simulink model "prosjektoppgave"  (R2026a)
settings: Solver=VariableStepAuto  StopTime=100
values from neighbouring files (symbols this model uses):
  A = pi*(r)^2    (= 0.785398163397)    [linearsimple.m]
  At = pi*(rt)^2    (= 0.0176714586764)    [linearsimple.m]
  Atut = At/2    (= 0.00883572933822)    [linearsimple.m]
  g = 9.80665    [linearsimple.m]
  gammaverdi = -0.025    [linearsimple.m]
  h = 1    [linearsimple.m]
  h10 = 0.8*h    (= 0.8)    [linearsimple.m]
  h20 = 0.5*h    (= 0.5)    [linearsimple.m]
  hf = 0*h    (= 0)    [linearsimple.m]
  href = 0.7    [linearsimple.m]
  Kd = (2*zeta*omega_0+gamma-a)/d    [linearsimple.m]
  Ki = gamma*omega_0^2/d    [linearsimple.m]
  Kp = (omega_0^2+2*gamma*zeta*omega_0-b)/d    [linearsimple.m]
  L = 0.1    [linearsimple.m]
  n = 2    [linearsimple.m]
  omega_0 = 0.4    [linearsimple.m]
  p = 1000    [linearsimple.m]
  r = 0.5    [linearsimple.m]
  rt = 0.075    [linearsimple.m]
  sin_Amp = sqrt(2*g*h)*At/(n*A)    [linearsimple.m]
  Tau = (sqrt(0.11)+L)*sqrt(2*h/g)    [linearsimple.m]
  zeta = 1    [linearsimple.m]
libraries: sl_discontinuities x15, simulink x5, vrlib x1
settings Model: PacingRate=5  Creator=User  LastModifiedBy=User

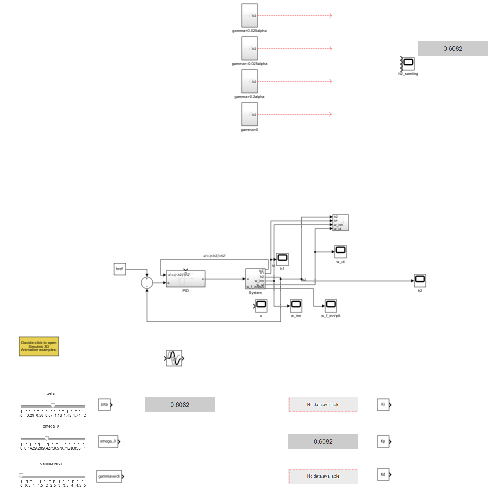
[thumbnail: Simulink's stored preview of the top-level diagram]
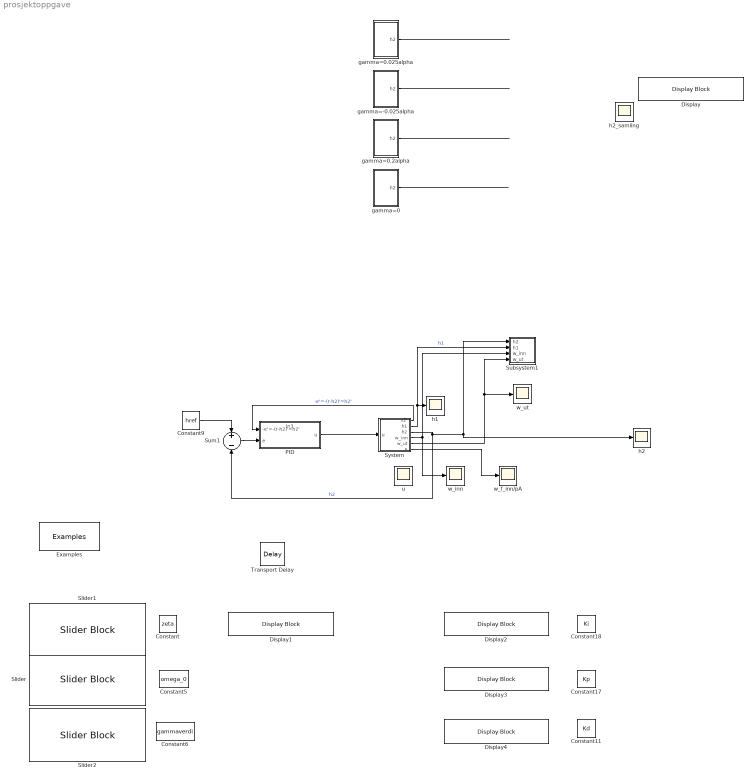
== system prosjektoppgave ==
  Constant : Constant  Value=zeta
  Constant11 : Constant  Value=Kd
  Constant17 : Constant  Value=Kp
  Constant18 : Constant  Value=Ki
  Constant5 : Constant  Value=omega_0
  Constant6 : Constant  Value=gammaverdi
  Constant9 : Constant  Value=href
  Display{,1..4} (5 alike) : DisplayBlock  LabelPosition=Hide  Transparency=1  GridColor=[0.502, 0.502, 0.502]
  Examples : vrlib/Examples
  PID : Subsystem
      settings: PortSchema="{\"entries\":[{\"content\":{\"sides\":[{\"content\":{\"connectorIds\":[\"In1\",\"In2\"]},\"type\":\"ConnectorPlacement.EquallySpacedRectSide\",\"uuid\":\"a96bb270-c3ec-4d15-9d6f-f29e3225f3c7\"},{\"content\":{\"connectorIds\":[\"Out1\"],\"side\":\"RIGHT\"},\"type\":\"ConnectorPlacement.EquallySpacedRectSide\",\"uuid\":\"f81bc953-5898-4b84-af0e-e30d44fc4639\"},{\"content\":{\"connectorIds\":[\"In3\"],\"side\":\"TOP\"},\"type\":\"ConnectorPlacement.EquallySpacedRectSide\",\"uuid\":\"08859213-698d-4bac-9d9f-733d026c3d6d\"}]},\"type\":\"ConnectorPlacement.EquallySpacedConnector\",\"uuid\":\"f15bc02d-61e9-4385-84d3-03e59a963aad\"}],\"packageUris\":[\"http://schema.mathworks.com/mf0/Connector/R2020b\"],\"version\":\"1.0\"}"
  Slider : SliderBlock  ScaleMax=1
  Slider1 : SliderBlock  ScaleMax=2
  Slider2 : SliderBlock  ScaleMax=5
  Subsystem1 : Subsystem
  Sum1 : Sum  Inputs=+-
  System : Subsystem
  Transport Delay : TransportDelay  DelayTime=Tau
  gamma=-0.025alpha : Subsystem
  gamma=0 : Subsystem
  gamma=0.025alpha : Subsystem
  gamma=0.2alpha : Subsystem
  h1 : Scope
      settings: ActiveDisplayYMinimum=0.74477697248915231  ActiveDisplayYMaximum=0.94477697248915227  DataLoggingVariableName=ScopeData6  DataLoggingSaveFormat=Array
  h2 : Scope
      settings: ActiveDisplayYMinimum=-0.00622784608789678  ActiveDisplayYMaximum=0.056050614791071034  DataLoggingVariableName=ScopeData11  DataLoggingSaveFormat=Array
  h2_samling : Scope  NumInputPorts=4
      settings: ActiveDisplayYMinimum=0.47019185858883861  ActiveDisplayYMaximum=0.76827327270045265  DataLoggingSaveFormat=Array
  u : Scope
      settings: ActiveDisplayYMinimum=-0.011988918852401206  ActiveDisplayYMaximum=0.078937646859600419  DataLoggingVariableName=ScopeData7  DataLoggingSaveFormat=Array
  w_f_inn/pA : Scope
      settings: ActiveDisplayYMinimum=-48.913386971378607  ActiveDisplayYMaximum=48.913374805426372  DataLoggingVariableName=ScopeData8  DataLoggingSaveFormat=Array
  w_inn : Scope
      settings: ActiveDisplayYMinimum=-9.7826777587122287  ActiveDisplayYMaximum=88.044099828410069  DataLoggingVariableName=ScopeData9  DataLoggingSaveFormat=Array
  w_ut : Scope
      settings: ActiveDisplayYMinimum=-0.00622784608789678  ActiveDisplayYMaximum=0.056050614791071034  DataLoggingVariableName=ScopeData10  DataLoggingSaveFormat=Array
  wires:
  gamma=0.025alpha/1(h2) -> ?
  gamma=-0.025alpha/1(h2) -> ?
  gamma=0.2alpha/1(h2) -> ?
  gamma=0/1(h2) -> ?
  System/4(w_inn) -> w_inn/1, Subsystem1/3(w_inn)
  Constant9/1 -> Sum1/1
  System/3(h2) -> h2/1, Subsystem1/1(h2), Sum1/2  "h2"
  System/2(h1) -> Subsystem1/2(h1), h1/1  "h1"
  System/5(w_ut) -> Subsystem1/4(w_ut), w_ut/1
  PID/1(u) -> System/1(u)
  System/6(w_f_inn/pA) -> w_f_inn/pA/1
  Sum1/1 -> PID/2(e)
  System/1(h2') -> PID/1(-e'=-(r-h2)'=h2')  "-e'=-(r-h2)'=h2'"

== system prosjektoppgave/PID ==
  -e'=-(r-h2)'=h2' : Inport
  e : Inport  Port=2
  In3 : Inport  Port=3
  Gain : Gain  Gain=1.2997
  Gain1 : Gain  Gain=-4.5681
  Gain2 : Gain  Gain=0.0126
  Integrator : Integrator
  Sum : Sum  Inputs=+++
  u : Outport
  wires:
  Integrator/1 -> Gain2/1
  Gain/1 -> Sum/2
  e/1 -> Gain/1, Integrator/1
  Gain2/1 -> Sum/3
  Gain1/1 -> Sum/1
  Sum/1 -> u/1
  -e'=-(r-h2)'=h2'/1 -> Gain1/1

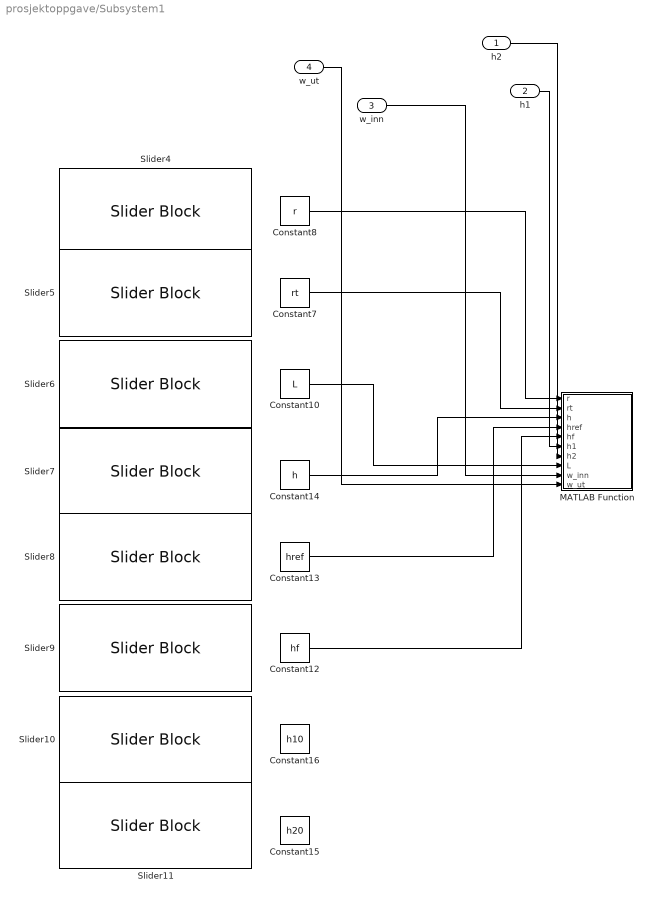
== system prosjektoppgave/Subsystem1 ==
  h2 : Inport
  h1 : Inport  Port=2
  w_inn : Inport  Port=3
  w_ut : Inport  Port=4
  Constant10 : Constant  Value=L
  Constant12 : Constant  Value=hf
  Constant13 : Constant  Value=href
  Constant14 : Constant  Value=h
  Constant15 : Constant  Value=h20
  Constant16 : Constant  Value=h10
  Constant7 : Constant  Value=rt
  Constant8 : Constant  Value=r
  MATLAB Function : MATLAB Function  TreatAsAtomicUnit=on
  Slider{4..5,10..11} (4 alike) : SliderBlock
  Slider{6..9} (4 alike) : SliderBlock  ScaleMax=1
  wires:
  h2/1 -> MATLAB Function/7(h2)
  Constant13/1 -> MATLAB Function/4(href)
  Constant10/1 -> MATLAB Function/8(L)
  Constant14/1 -> MATLAB Function/3(h)
  h1/1 -> MATLAB Function/6(h1)
  Constant12/1 -> MATLAB Function/5(hf)
  Constant8/1 -> MATLAB Function/1(r)
  Constant7/1 -> MATLAB Function/2(rt)
  w_inn/1 -> MATLAB Function/9(w_inn)
  w_ut/1 -> MATLAB Function/10(w_ut)

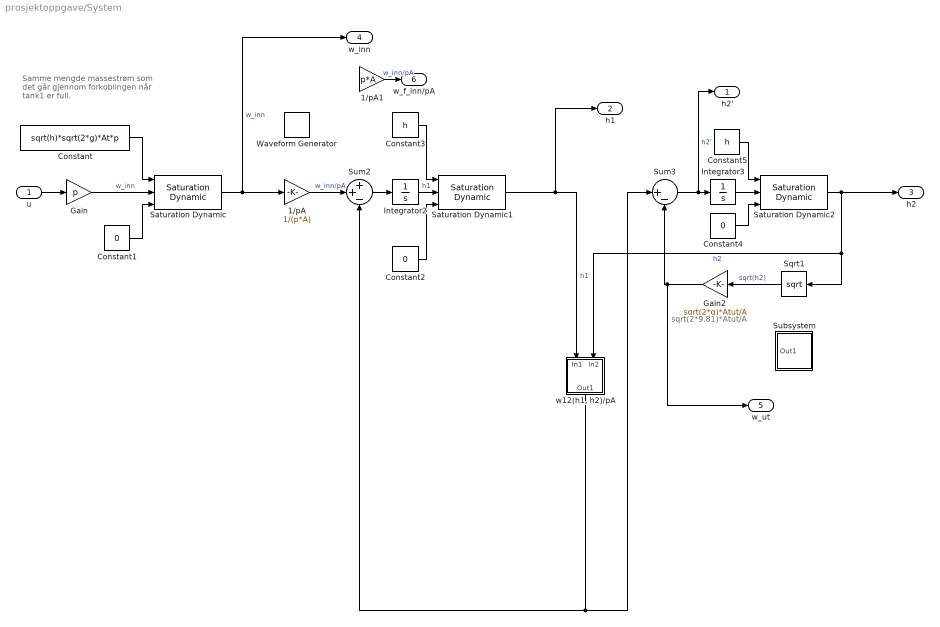
== system prosjektoppgave/System ==
  note: Samme mengde massestrøm
      | som det går gjennom
      | forkoblingen når tank1 er full.
  note: sqrt(2*9.81)*Atut/A
  u : Inport  OutMin=0
  1/pA : Gain  Gain=1/(p*A)
  1/pA1 : Gain  Gain=p*A
  Constant : Constant  Value=sqrt(h)*sqrt(2*g)*At*p
  Constant1 : Constant  Value=0
  Constant2 : Constant  Value=0
  Constant3 : Constant  Value=h
  Constant4 : Constant  Value=0
  Constant5 : Constant  Value=h
  Gain : Gain  Gain=p
  Gain2 : Gain  Gain=sqrt(2*g)*Atut/A
  Integrator2 : Integrator  InitialCondition=h10
  Integrator3 : Integrator  InitialCondition=h20
  Saturation Dynamic : sl_discontinuities/Saturation Dynamic  OutMin=[]  OutMax=[]  OutDataTypeStr=Inherit: Same as second input  OutDataType=fixdt(1, 16)  OutScaling=2^-10  DoSatur=off
      settings: LibrarySourceBlock=|
      | simulink/Discontinuities/Saturation
      | Dynamic
  Saturation Dynamic1 : sl_discontinuities/Saturation Dynamic  OutMin=[]  OutMax=[]  OutDataTypeStr=Inherit: Same as second input  OutDataType=fixdt(1, 16)  OutScaling=2^-10  DoSatur=off
      settings: LibrarySourceBlock=|
      | simulink/Discontinuities/Saturation
      | Dynamic
  Saturation Dynamic2 : sl_discontinuities/Saturation Dynamic  OutMin=[]  OutMax=[]  OutDataTypeStr=Inherit: Same as second input  OutDataType=fixdt(1, 16)  OutScaling=2^-10  DoSatur=off
      settings: LibrarySourceBlock=|
      | simulink/Discontinuities/Saturation
      | Dynamic
  Sqrt1 : Sqrt
  Subsystem : Subsystem
  Sum2 : Sum  Inputs=++-
  Sum3 : Sum  Inputs=|+-
  Waveform Generator : simulink/Sources/Waveform Generator  OutMin=0  OutMax=sqrt(2*g)*At/(n*A)  OutDataTypeStr=double  SelectedSignal=1  Signals=sin(sin_Amp, 0.025, 0)  BlockNames=MultiportSwitch_05447e85ab52467  SampleTime=0.1
  "w12(h1, h2)/pA" : Subsystem
  h2' : Outport  VectorParamsAs1DForOutWhenUnconnected=off
  h1 : Outport  Port=2
  h2 : Outport  Port=3
  w_inn : Outport  Port=4
  w_ut : Outport  Port=5
  w_f_inn/pA : Outport  Port=6
  wires:
  Sum2/1 -> Integrator2/1
  Sum3/1 -> h2'/1, Integrator3/1  "h2'"
  Constant1/1 -> Saturation Dynamic/3
  Constant/1 -> Saturation Dynamic/1
  Integrator2/1 -> Saturation Dynamic1/2  "h1"
  Saturation Dynamic1/1 -> "w12(h1, h2)/pA"/1(In1), h1/1  "h1"
  Constant2/1 -> Saturation Dynamic1/3
  Constant3/1 -> Saturation Dynamic1/1
  Integrator3/1 -> Saturation Dynamic2/2
  Saturation Dynamic2/1 -> Sqrt1/1, "w12(h1, h2)/pA"/2(In2), h2/1  "h2"
  Constant4/1 -> Saturation Dynamic2/3
  Constant5/1 -> Saturation Dynamic2/1
  u/1 -> Gain/1
  Gain/1 -> Saturation Dynamic/2  "w_inn"
  Saturation Dynamic/1 -> w_inn/1, 1/pA/1  "w_inn"
  1/pA/1 -> Sum2/2  "w_inn/pA"
  ? -> 1/pA1/1, Sum2/1  "w_f_inn/pA"
  "w12(h1, h2)/pA"/1(Out1) -> Sum3/1, Sum2/3
  Sqrt1/1 -> Gain2/1  "sqrt(h2)"
  1/pA1/1 -> w_f_inn/pA/1  "w_inn/pA"
  Gain2/1 -> w_ut/1, Sum3/2

== system prosjektoppgave/gamma=-0.025alpha ==
  Constant9 : Constant  Value=href
  PID : Subsystem
  Subsystem1 : Subsystem
  Sum1 : Sum  Inputs=+-
  System : Subsystem
  h1 : Scope
      settings: ActiveDisplayYMinimum=0.74477697248915231  ActiveDisplayYMaximum=0.94477697248915227  DataLoggingVariableName=ScopeData2  DataLoggingSaveFormat=Array
  u : Scope
      settings: ActiveDisplayYMinimum=-0.011988918852401206  ActiveDisplayYMaximum=0.078937646859600419  DataLoggingVariableName=ScopeData4  DataLoggingSaveFormat=Array
  w_f_inn/pA : Scope
      settings: ActiveDisplayYMinimum=-48.913386971378607  ActiveDisplayYMaximum=48.913374805426372  DataLoggingVariableName=ScopeData5  DataLoggingSaveFormat=Array
  w_inn : Scope
      settings: ActiveDisplayYMinimum=-9.7826777587122287  ActiveDisplayYMaximum=88.044099828410069  DataLoggingSaveFormat=Array
  w_ut : Scope
      settings: ActiveDisplayYMinimum=-0.00622784608789678  ActiveDisplayYMaximum=0.056050614791071034  DataLoggingVariableName=ScopeData3  DataLoggingSaveFormat=Array
  h2 : Outport
  wires:
  System/3(h2) -> h2/1, Subsystem1/1(h2), Sum1/2  "h2"
  System/4(w_inn) -> w_inn/1, Subsystem1/3(w_inn)
  System/5(w_ut) -> Subsystem1/4(w_ut), w_ut/1
  System/2(h1) -> Subsystem1/2(h1), h1/1  "h1"
  Sum1/1 -> PID/2(e)
  Constant9/1 -> Sum1/1
  System/1(h2') -> PID/1(-e'=-(r-h2)'=h2')  "-e'=-(r-h2)'=h2'"
  System/6(w_f_inn/pA) -> w_f_inn/pA/1
  PID/1(u) -> System/1(u)

== system prosjektoppgave/gamma=0 ==
  Constant9 : Constant  Value=href
  PID : Subsystem
  Subsystem1 : Subsystem
  Sum1 : Sum  Inputs=+-
  System : Subsystem
  h1 : Scope
      settings: ActiveDisplayYMinimum=0.74477697248915231  ActiveDisplayYMaximum=0.94477697248915227  DataLoggingVariableName=ScopeData2  DataLoggingSaveFormat=Array
  u : Scope
      settings: ActiveDisplayYMinimum=-0.011988918852401206  ActiveDisplayYMaximum=0.078937646859600419  DataLoggingVariableName=ScopeData4  DataLoggingSaveFormat=Array
  w_f_inn/pA : Scope
      settings: ActiveDisplayYMinimum=-48.913386971378607  ActiveDisplayYMaximum=48.913374805426372  DataLoggingVariableName=ScopeData5  DataLoggingSaveFormat=Array
  w_inn : Scope
      settings: ActiveDisplayYMinimum=-9.7826777587122287  ActiveDisplayYMaximum=88.044099828410069  DataLoggingSaveFormat=Array
  w_ut : Scope
      settings: ActiveDisplayYMinimum=-0.00622784608789678  ActiveDisplayYMaximum=0.056050614791071034  DataLoggingVariableName=ScopeData3  DataLoggingSaveFormat=Array
  h2 : Outport
  wires:
  System/3(h2) -> h2/1, Subsystem1/1(h2), Sum1/2  "h2"
  System/4(w_inn) -> w_inn/1, Subsystem1/3(w_inn)
  System/5(w_ut) -> Subsystem1/4(w_ut), w_ut/1
  System/2(h1) -> Subsystem1/2(h1), h1/1  "h1"
  Sum1/1 -> PID/2(e)
  Constant9/1 -> Sum1/1
  System/1(h2') -> PID/1(-e'=-(r-h2)'=h2')  "-e'=-(r-h2)'=h2'"
  System/6(w_f_inn/pA) -> w_f_inn/pA/1
  PID/1(u) -> System/1(u)

== system prosjektoppgave/gamma=0.025alpha ==
  Constant9 : Constant  Value=href
  PID : Subsystem
  Subsystem1 : Subsystem
  Sum1 : Sum  Inputs=+-
  System : Subsystem
  h1 : Scope
      settings: ActiveDisplayYMinimum=0.74477697248915231  ActiveDisplayYMaximum=0.94477697248915227  DataLoggingVariableName=ScopeData2  DataLoggingSaveFormat=Array
  u : Scope
      settings: ActiveDisplayYMinimum=-0.011988918852401206  ActiveDisplayYMaximum=0.078937646859600419  DataLoggingVariableName=ScopeData4  DataLoggingSaveFormat=Array
  w_f_inn/pA : Scope
      settings: ActiveDisplayYMinimum=-48.913386971378607  ActiveDisplayYMaximum=48.913374805426372  DataLoggingVariableName=ScopeData5  DataLoggingSaveFormat=Array
  w_inn : Scope
      settings: ActiveDisplayYMinimum=-9.7826777587122287  ActiveDisplayYMaximum=88.044099828410069  DataLoggingSaveFormat=Array
  w_ut : Scope
      settings: ActiveDisplayYMinimum=-0.00622784608789678  ActiveDisplayYMaximum=0.056050614791071034  DataLoggingVariableName=ScopeData3  DataLoggingSaveFormat=Array
  h2 : Outport
  wires:
  System/3(h2) -> h2/1, Subsystem1/1(h2), Sum1/2  "h2"
  System/4(w_inn) -> w_inn/1, Subsystem1/3(w_inn)
  System/5(w_ut) -> Subsystem1/4(w_ut), w_ut/1
  System/2(h1) -> Subsystem1/2(h1), h1/1  "h1"
  Sum1/1 -> PID/2(e)
  Constant9/1 -> Sum1/1
  System/1(h2') -> PID/1(-e'=-(r-h2)'=h2')  "-e'=-(r-h2)'=h2'"
  System/6(w_f_inn/pA) -> w_f_inn/pA/1
  PID/1(u) -> System/1(u)

== system prosjektoppgave/gamma=0.2alpha ==
  Constant9 : Constant  Value=href
  PID : Subsystem
  Subsystem1 : Subsystem
  Sum1 : Sum  Inputs=+-
  System : Subsystem
  h1 : Scope
      settings: ActiveDisplayYMinimum=0.74477697248915231  ActiveDisplayYMaximum=0.94477697248915227  DataLoggingVariableName=ScopeData2  DataLoggingSaveFormat=Array
  u : Scope
      settings: ActiveDisplayYMinimum=-0.011988918852401206  ActiveDisplayYMaximum=0.078937646859600419  DataLoggingVariableName=ScopeData4  DataLoggingSaveFormat=Array
  w_f_inn/pA : Scope
      settings: ActiveDisplayYMinimum=-48.913386971378607  ActiveDisplayYMaximum=48.913374805426372  DataLoggingVariableName=ScopeData5  DataLoggingSaveFormat=Array
  w_inn : Scope
      settings: ActiveDisplayYMinimum=-9.7826777587122287  ActiveDisplayYMaximum=88.044099828410069  DataLoggingSaveFormat=Array
  w_ut : Scope
      settings: ActiveDisplayYMinimum=-0.00622784608789678  ActiveDisplayYMaximum=0.056050614791071034  DataLoggingVariableName=ScopeData3  DataLoggingSaveFormat=Array
  h2 : Outport
  wires:
  System/3(h2) -> h2/1, Subsystem1/1(h2), Sum1/2  "h2"
  System/4(w_inn) -> w_inn/1, Subsystem1/3(w_inn)
  System/5(w_ut) -> Subsystem1/4(w_ut), w_ut/1
  System/2(h1) -> Subsystem1/2(h1), h1/1  "h1"
  Sum1/1 -> PID/2(e)
  Constant9/1 -> Sum1/1
  System/1(h2') -> PID/1(-e'=-(r-h2)'=h2')  "-e'=-(r-h2)'=h2'"
  System/6(w_f_inn/pA) -> w_f_inn/pA/1
  PID/1(u) -> System/1(u)

== system prosjektoppgave/System/Subsystem ==
  Constant1 : Constant  Value=0
  Constant2 : Constant  Value=sqrt(2*g)*Atut*sqrt(h)/A
  Switch : Switch  Threshold=5  SaturateOnIntegerOverflow=off  InputSameDT=off
  Uniform Random Number : UniformRandomNumber  Minimum=0  Maximum=10  SampleTime=20
  Out1 : Outport
  wires:
  Uniform Random Number/1 -> Switch/2
  Switch/1 -> Out1/1
  Constant1/1 -> Switch/1
  Constant2/1 -> Switch/3

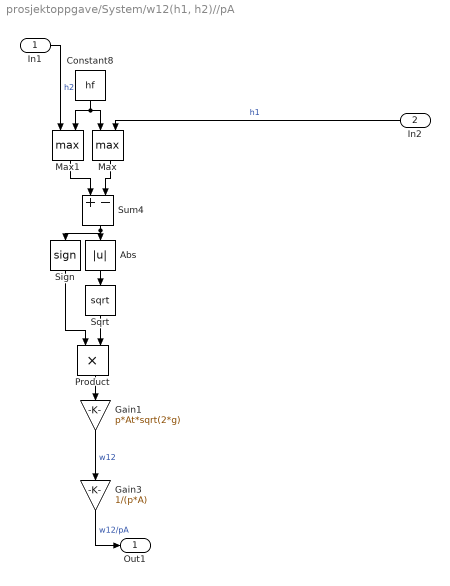
== system prosjektoppgave/System/w12(h1, h2)//pA ==
  In1 : Inport
  In2 : Inport  Port=2
  Abs : Abs  SaturateOnIntegerOverflow=off
  Constant8 : Constant  Value=hf
  Gain1 : Gain  Gain=p*At*sqrt(2*g)
  Gain3 : Gain  Gain=1/(p*A)
  Max : MinMax  Function=max  Inputs=2
  Max1 : MinMax  Function=max  Inputs=2
  Product : Product
  Sign : Signum
  Sqrt : Sqrt
  Sum4 : Sum  Inputs=+-
  Out1 : Outport
  wires:
  Constant8/1 -> Max1/2, Max/1
  Sum4/1 -> Sign/1, Abs/1
  Max1/1 -> Sum4/1
  Max/1 -> Sum4/2
  Product/1 -> Gain1/1
  Sqrt/1 -> Product/2
  In1/1 -> Max1/1  "h2"
  Sign/1 -> Product/1
  Abs/1 -> Sqrt/1
  Gain1/1 -> Gain3/1  "w12"
  In2/1 -> Max/2  "h1"
  Gain3/1 -> Out1/1  "w12/pA"

== system prosjektoppgave/gamma=-0.025alpha/PID ==
  -e'=-(r-h2)'=h2' : Inport
  e : Inport  Port=2
  Gain : Gain  Gain=Kp
  Gain1 : Gain  Gain=-Kd
  Gain2 : Gain  Gain=Ki
  Integrator : Integrator
  Sum : Sum  Inputs=+++
  u : Outport
  wires:
  Integrator/1 -> Gain2/1
  Gain/1 -> Sum/2
  e/1 -> Gain/1, Integrator/1
  Gain2/1 -> Sum/3
  Gain1/1 -> Sum/1
  Sum/1 -> u/1
  -e'=-(r-h2)'=h2'/1 -> Gain1/1

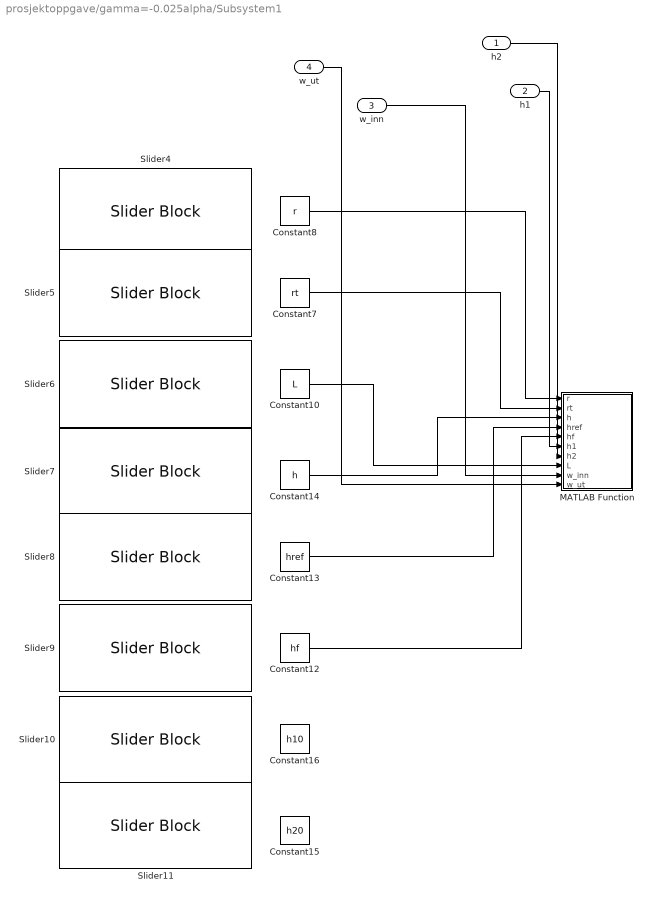
== system prosjektoppgave/gamma=-0.025alpha/Subsystem1 ==
  h2 : Inport
  h1 : Inport  Port=2
  w_inn : Inport  Port=3
  w_ut : Inport  Port=4
  Constant10 : Constant  Value=L
  Constant12 : Constant  Value=hf
  Constant13 : Constant  Value=href
  Constant14 : Constant  Value=h
  Constant15 : Constant  Value=h20
  Constant16 : Constant  Value=h10
  Constant7 : Constant  Value=rt
  Constant8 : Constant  Value=r
  MATLAB Function : MATLAB Function  TreatAsAtomicUnit=on
  Slider{4..5,10..11} (4 alike) : SliderBlock
  Slider{6..9} (4 alike) : SliderBlock  ScaleMax=1
  wires:
  h2/1 -> MATLAB Function/7(h2)
  Constant13/1 -> MATLAB Function/4(href)
  Constant10/1 -> MATLAB Function/8(L)
  Constant14/1 -> MATLAB Function/3(h)
  h1/1 -> MATLAB Function/6(h1)
  Constant12/1 -> MATLAB Function/5(hf)
  Constant8/1 -> MATLAB Function/1(r)
  Constant7/1 -> MATLAB Function/2(rt)
  w_inn/1 -> MATLAB Function/9(w_inn)
  w_ut/1 -> MATLAB Function/10(w_ut)

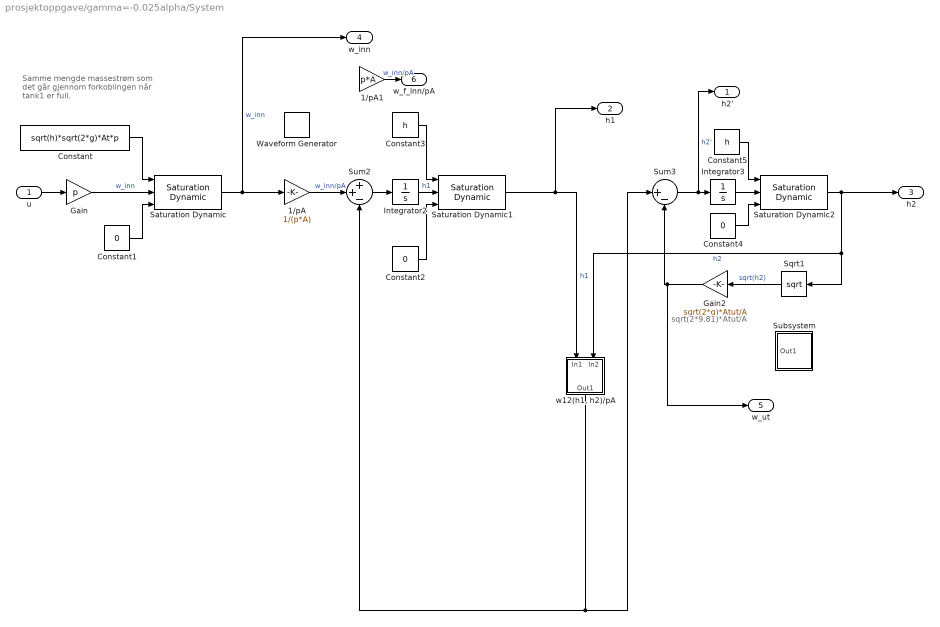
== system prosjektoppgave/gamma=-0.025alpha/System ==
  note: Samme mengde massestrøm
      | som det går gjennom
      | forkoblingen når tank1 er full.
  note: sqrt(2*9.81)*Atut/A
  u : Inport  OutMin=0
  1/pA : Gain  Gain=1/(p*A)
  1/pA1 : Gain  Gain=p*A
  Constant : Constant  Value=sqrt(h)*sqrt(2*g)*At*p
  Constant1 : Constant  Value=0
  Constant2 : Constant  Value=0
  Constant3 : Constant  Value=h
  Constant4 : Constant  Value=0
  Constant5 : Constant  Value=h
  Gain : Gain  Gain=p
  Gain2 : Gain  Gain=sqrt(2*g)*Atut/A
  Integrator2 : Integrator  InitialCondition=h10
  Integrator3 : Integrator  InitialCondition=h20
  Saturation Dynamic : sl_discontinuities/Saturation Dynamic  OutMin=[]  OutMax=[]  OutDataTypeStr=Inherit: Same as second input  OutDataType=fixdt(1, 16)  OutScaling=2^-10  DoSatur=off
      settings: LibrarySourceBlock=|
      | simulink/Discontinuities/Saturation
      | Dynamic
  Saturation Dynamic1 : sl_discontinuities/Saturation Dynamic  OutMin=[]  OutMax=[]  OutDataTypeStr=Inherit: Same as second input  OutDataType=fixdt(1, 16)  OutScaling=2^-10  DoSatur=off
      settings: LibrarySourceBlock=|
      | simulink/Discontinuities/Saturation
      | Dynamic
  Saturation Dynamic2 : sl_discontinuities/Saturation Dynamic  OutMin=[]  OutMax=[]  OutDataTypeStr=Inherit: Same as second input  OutDataType=fixdt(1, 16)  OutScaling=2^-10  DoSatur=off
      settings: LibrarySourceBlock=|
      | simulink/Discontinuities/Saturation
      | Dynamic
  Sqrt1 : Sqrt
  Subsystem : Subsystem
  Sum2 : Sum  Inputs=++-
  Sum3 : Sum  Inputs=|+-
  Waveform Generator : simulink/Sources/Waveform Generator  OutMin=0  OutMax=sqrt(2*g)*At/(n*A)  OutDataTypeStr=double  SelectedSignal=1  Signals=sin(sin_Amp, 0.025, 0)  BlockNames=MultiportSwitch_05447e85ab52467  SampleTime=0.1
  "w12(h1, h2)/pA" : Subsystem
  h2' : Outport  VectorParamsAs1DForOutWhenUnconnected=off
  h1 : Outport  Port=2
  h2 : Outport  Port=3
  w_inn : Outport  Port=4
  w_ut : Outport  Port=5
  w_f_inn/pA : Outport  Port=6
  wires:
  Sum2/1 -> Integrator2/1
  Sum3/1 -> h2'/1, Integrator3/1  "h2'"
  Constant1/1 -> Saturation Dynamic/3
  Constant/1 -> Saturation Dynamic/1
  Integrator2/1 -> Saturation Dynamic1/2  "h1"
  Saturation Dynamic1/1 -> "w12(h1, h2)/pA"/1(In1), h1/1  "h1"
  Constant2/1 -> Saturation Dynamic1/3
  Constant3/1 -> Saturation Dynamic1/1
  Integrator3/1 -> Saturation Dynamic2/2
  Saturation Dynamic2/1 -> Sqrt1/1, "w12(h1, h2)/pA"/2(In2), h2/1  "h2"
  Constant4/1 -> Saturation Dynamic2/3
  Constant5/1 -> Saturation Dynamic2/1
  u/1 -> Gain/1
  Gain/1 -> Saturation Dynamic/2  "w_inn"
  Saturation Dynamic/1 -> w_inn/1, 1/pA/1  "w_inn"
  1/pA/1 -> Sum2/2  "w_inn/pA"
  ? -> 1/pA1/1, Sum2/1  "w_f_inn/pA"
  "w12(h1, h2)/pA"/1(Out1) -> Sum3/1, Sum2/3
  Sqrt1/1 -> Gain2/1  "sqrt(h2)"
  1/pA1/1 -> w_f_inn/pA/1  "w_inn/pA"
  Gain2/1 -> w_ut/1, Sum3/2

== system prosjektoppgave/gamma=0/PID ==
  -e'=-(r-h2)'=h2' : Inport
  e : Inport  Port=2
  Gain : Gain  Gain=1.2367
  Gain1 : Gain  Gain=-4.4893
  Gain2 : Gain  Gain=0
  Integrator : Integrator
  Sum : Sum  Inputs=+++
  u : Outport
  wires:
  Integrator/1 -> Gain2/1
  Gain/1 -> Sum/2
  e/1 -> Gain/1, Integrator/1
  Gain2/1 -> Sum/3
  Gain1/1 -> Sum/1
  Sum/1 -> u/1
  -e'=-(r-h2)'=h2'/1 -> Gain1/1

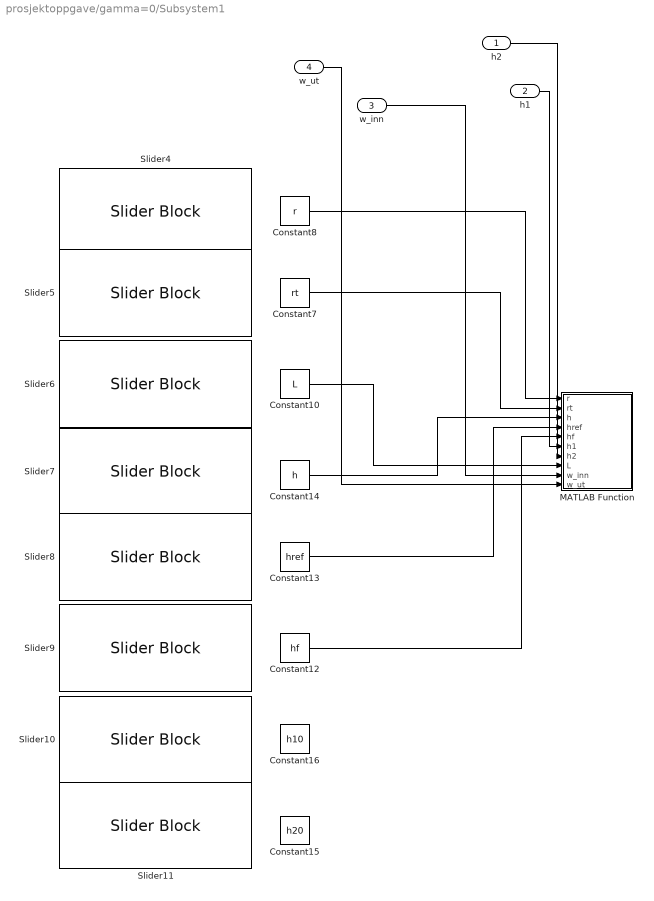
== system prosjektoppgave/gamma=0/Subsystem1 ==
  h2 : Inport
  h1 : Inport  Port=2
  w_inn : Inport  Port=3
  w_ut : Inport  Port=4
  Constant10 : Constant  Value=L
  Constant12 : Constant  Value=hf
  Constant13 : Constant  Value=href
  Constant14 : Constant  Value=h
  Constant15 : Constant  Value=h20
  Constant16 : Constant  Value=h10
  Constant7 : Constant  Value=rt
  Constant8 : Constant  Value=r
  MATLAB Function : MATLAB Function  TreatAsAtomicUnit=on
  Slider{4..5,10..11} (4 alike) : SliderBlock
  Slider{6..9} (4 alike) : SliderBlock  ScaleMax=1
  wires:
  h2/1 -> MATLAB Function/7(h2)
  Constant13/1 -> MATLAB Function/4(href)
  Constant10/1 -> MATLAB Function/8(L)
  Constant14/1 -> MATLAB Function/3(h)
  h1/1 -> MATLAB Function/6(h1)
  Constant12/1 -> MATLAB Function/5(hf)
  Constant8/1 -> MATLAB Function/1(r)
  Constant7/1 -> MATLAB Function/2(rt)
  w_inn/1 -> MATLAB Function/9(w_inn)
  w_ut/1 -> MATLAB Function/10(w_ut)

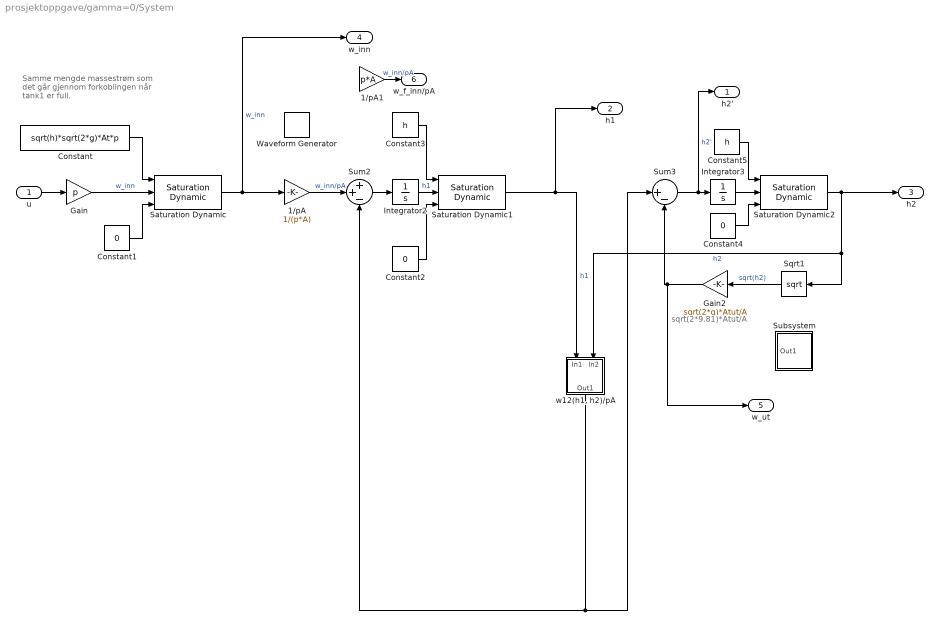
== system prosjektoppgave/gamma=0/System ==
  note: Samme mengde massestrøm
      | som det går gjennom
      | forkoblingen når tank1 er full.
  note: sqrt(2*9.81)*Atut/A
  u : Inport  OutMin=0
  1/pA : Gain  Gain=1/(p*A)
  1/pA1 : Gain  Gain=p*A
  Constant : Constant  Value=sqrt(h)*sqrt(2*g)*At*p
  Constant1 : Constant  Value=0
  Constant2 : Constant  Value=0
  Constant3 : Constant  Value=h
  Constant4 : Constant  Value=0
  Constant5 : Constant  Value=h
  Gain : Gain  Gain=p
  Gain2 : Gain  Gain=sqrt(2*g)*Atut/A
  Integrator2 : Integrator  InitialCondition=h10
  Integrator3 : Integrator  InitialCondition=h20
  Saturation Dynamic : sl_discontinuities/Saturation Dynamic  OutMin=[]  OutMax=[]  OutDataTypeStr=Inherit: Same as second input  OutDataType=fixdt(1, 16)  OutScaling=2^-10  DoSatur=off
      settings: LibrarySourceBlock=|
      | simulink/Discontinuities/Saturation
      | Dynamic
  Saturation Dynamic1 : sl_discontinuities/Saturation Dynamic  OutMin=[]  OutMax=[]  OutDataTypeStr=Inherit: Same as second input  OutDataType=fixdt(1, 16)  OutScaling=2^-10  DoSatur=off
      settings: LibrarySourceBlock=|
      | simulink/Discontinuities/Saturation
      | Dynamic
  Saturation Dynamic2 : sl_discontinuities/Saturation Dynamic  OutMin=[]  OutMax=[]  OutDataTypeStr=Inherit: Same as second input  OutDataType=fixdt(1, 16)  OutScaling=2^-10  DoSatur=off
      settings: LibrarySourceBlock=|
      | simulink/Discontinuities/Saturation
      | Dynamic
  Sqrt1 : Sqrt
  Subsystem : Subsystem
  Sum2 : Sum  Inputs=++-
  Sum3 : Sum  Inputs=|+-
  Waveform Generator : simulink/Sources/Waveform Generator  OutMin=0  OutMax=sqrt(2*g)*At/(n*A)  OutDataTypeStr=double  SelectedSignal=1  Signals=sin(sin_Amp, 0.025, 0)  BlockNames=MultiportSwitch_05447e85ab52467  SampleTime=0.1
  "w12(h1, h2)/pA" : Subsystem
  h2' : Outport  VectorParamsAs1DForOutWhenUnconnected=off
  h1 : Outport  Port=2
  h2 : Outport  Port=3
  w_inn : Outport  Port=4
  w_ut : Outport  Port=5
  w_f_inn/pA : Outport  Port=6
  wires:
  Sum2/1 -> Integrator2/1
  Sum3/1 -> h2'/1, Integrator3/1  "h2'"
  Constant1/1 -> Saturation Dynamic/3
  Constant/1 -> Saturation Dynamic/1
  Integrator2/1 -> Saturation Dynamic1/2  "h1"
  Saturation Dynamic1/1 -> "w12(h1, h2)/pA"/1(In1), h1/1  "h1"
  Constant2/1 -> Saturation Dynamic1/3
  Constant3/1 -> Saturation Dynamic1/1
  Integrator3/1 -> Saturation Dynamic2/2
  Saturation Dynamic2/1 -> Sqrt1/1, "w12(h1, h2)/pA"/2(In2), h2/1  "h2"
  Constant4/1 -> Saturation Dynamic2/3
  Constant5/1 -> Saturation Dynamic2/1
  u/1 -> Gain/1
  Gain/1 -> Saturation Dynamic/2  "w_inn"
  Saturation Dynamic/1 -> w_inn/1, 1/pA/1  "w_inn"
  1/pA/1 -> Sum2/2  "w_inn/pA"
  ? -> 1/pA1/1, Sum2/1  "w_f_inn/pA"
  "w12(h1, h2)/pA"/1(Out1) -> Sum3/1, Sum2/3
  Sqrt1/1 -> Gain2/1  "sqrt(h2)"
  1/pA1/1 -> w_f_inn/pA/1  "w_inn/pA"
  Gain2/1 -> w_ut/1, Sum3/2

== system prosjektoppgave/gamma=0.025alpha/PID ==
  -e'=-(r-h2)'=h2' : Inport
  e : Inport  Port=2
  Gain : Gain  Gain=1.2997
  Gain1 : Gain  Gain=-4.5681
  Gain2 : Gain  Gain=0.0126
  Integrator : Integrator
  Sum : Sum  Inputs=+++
  u : Outport
  wires:
  Integrator/1 -> Gain2/1
  Gain/1 -> Sum/2
  e/1 -> Gain/1, Integrator/1
  Gain2/1 -> Sum/3
  Gain1/1 -> Sum/1
  Sum/1 -> u/1
  -e'=-(r-h2)'=h2'/1 -> Gain1/1

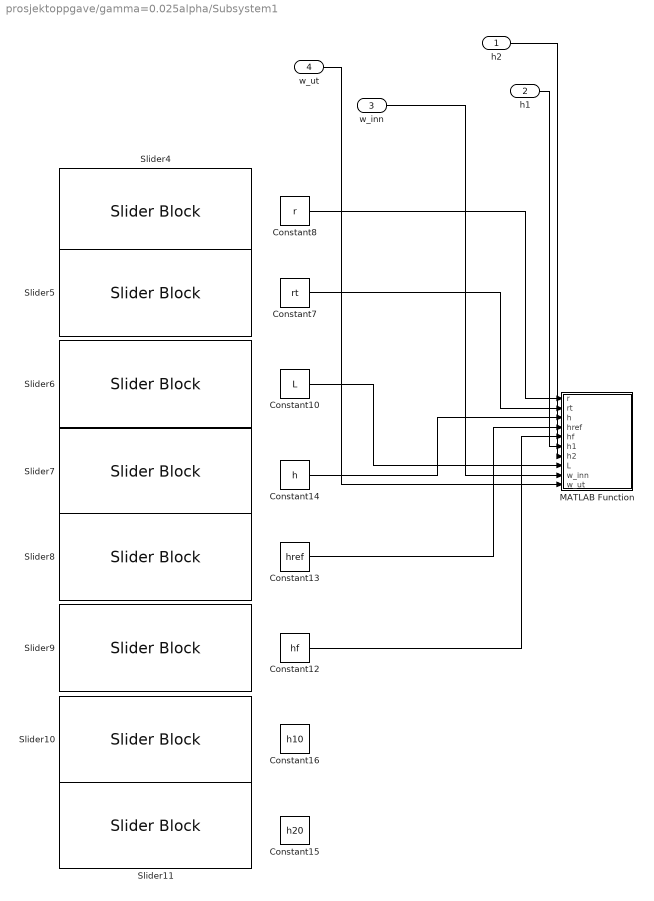
== system prosjektoppgave/gamma=0.025alpha/Subsystem1 ==
  h2 : Inport
  h1 : Inport  Port=2
  w_inn : Inport  Port=3
  w_ut : Inport  Port=4
  Constant10 : Constant  Value=L
  Constant12 : Constant  Value=hf
  Constant13 : Constant  Value=href
  Constant14 : Constant  Value=h
  Constant15 : Constant  Value=h20
  Constant16 : Constant  Value=h10
  Constant7 : Constant  Value=rt
  Constant8 : Constant  Value=r
  MATLAB Function : MATLAB Function  TreatAsAtomicUnit=on
  Slider{4..5,10..11} (4 alike) : SliderBlock
  Slider{6..9} (4 alike) : SliderBlock  ScaleMax=1
  wires:
  h2/1 -> MATLAB Function/7(h2)
  Constant13/1 -> MATLAB Function/4(href)
  Constant10/1 -> MATLAB Function/8(L)
  Constant14/1 -> MATLAB Function/3(h)
  h1/1 -> MATLAB Function/6(h1)
  Constant12/1 -> MATLAB Function/5(hf)
  Constant8/1 -> MATLAB Function/1(r)
  Constant7/1 -> MATLAB Function/2(rt)
  w_inn/1 -> MATLAB Function/9(w_inn)
  w_ut/1 -> MATLAB Function/10(w_ut)

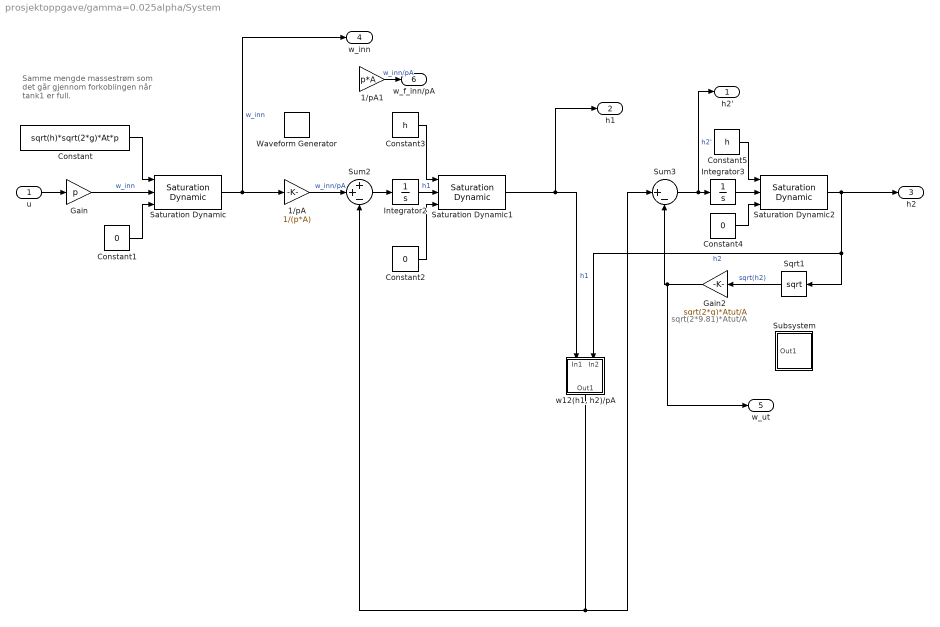
== system prosjektoppgave/gamma=0.025alpha/System ==
  note: Samme mengde massestrøm
      | som det går gjennom
      | forkoblingen når tank1 er full.
  note: sqrt(2*9.81)*Atut/A
  u : Inport  OutMin=0
  1/pA : Gain  Gain=1/(p*A)
  1/pA1 : Gain  Gain=p*A
  Constant : Constant  Value=sqrt(h)*sqrt(2*g)*At*p
  Constant1 : Constant  Value=0
  Constant2 : Constant  Value=0
  Constant3 : Constant  Value=h
  Constant4 : Constant  Value=0
  Constant5 : Constant  Value=h
  Gain : Gain  Gain=p
  Gain2 : Gain  Gain=sqrt(2*g)*Atut/A
  Integrator2 : Integrator  InitialCondition=h10
  Integrator3 : Integrator  InitialCondition=h20
  Saturation Dynamic : sl_discontinuities/Saturation Dynamic  OutMin=[]  OutMax=[]  OutDataTypeStr=Inherit: Same as second input  OutDataType=fixdt(1, 16)  OutScaling=2^-10  DoSatur=off
      settings: LibrarySourceBlock=|
      | simulink/Discontinuities/Saturation
      | Dynamic
  Saturation Dynamic1 : sl_discontinuities/Saturation Dynamic  OutMin=[]  OutMax=[]  OutDataTypeStr=Inherit: Same as second input  OutDataType=fixdt(1, 16)  OutScaling=2^-10  DoSatur=off
      settings: LibrarySourceBlock=|
      | simulink/Discontinuities/Saturation
      | Dynamic
  Saturation Dynamic2 : sl_discontinuities/Saturation Dynamic  OutMin=[]  OutMax=[]  OutDataTypeStr=Inherit: Same as second input  OutDataType=fixdt(1, 16)  OutScaling=2^-10  DoSatur=off
      settings: LibrarySourceBlock=|
      | simulink/Discontinuities/Saturation
      | Dynamic
  Sqrt1 : Sqrt
  Subsystem : Subsystem
  Sum2 : Sum  Inputs=++-
  Sum3 : Sum  Inputs=|+-
  Waveform Generator : simulink/Sources/Waveform Generator  OutMin=0  OutMax=sqrt(2*g)*At/(n*A)  OutDataTypeStr=double  SelectedSignal=1  Signals=sin(sin_Amp, 0.025, 0)  BlockNames=MultiportSwitch_05447e85ab52467  SampleTime=0.1
  "w12(h1, h2)/pA" : Subsystem
  h2' : Outport  VectorParamsAs1DForOutWhenUnconnected=off
  h1 : Outport  Port=2
  h2 : Outport  Port=3
  w_inn : Outport  Port=4
  w_ut : Outport  Port=5
  w_f_inn/pA : Outport  Port=6
  wires:
  Sum2/1 -> Integrator2/1
  Sum3/1 -> h2'/1, Integrator3/1  "h2'"
  Constant1/1 -> Saturation Dynamic/3
  Constant/1 -> Saturation Dynamic/1
  Integrator2/1 -> Saturation Dynamic1/2  "h1"
  Saturation Dynamic1/1 -> "w12(h1, h2)/pA"/1(In1), h1/1  "h1"
  Constant2/1 -> Saturation Dynamic1/3
  Constant3/1 -> Saturation Dynamic1/1
  Integrator3/1 -> Saturation Dynamic2/2
  Saturation Dynamic2/1 -> Sqrt1/1, "w12(h1, h2)/pA"/2(In2), h2/1  "h2"
  Constant4/1 -> Saturation Dynamic2/3
  Constant5/1 -> Saturation Dynamic2/1
  u/1 -> Gain/1
  Gain/1 -> Saturation Dynamic/2  "w_inn"
  Saturation Dynamic/1 -> w_inn/1, 1/pA/1  "w_inn"
  1/pA/1 -> Sum2/2  "w_inn/pA"
  ? -> 1/pA1/1, Sum2/1  "w_f_inn/pA"
  "w12(h1, h2)/pA"/1(Out1) -> Sum3/1, Sum2/3
  Sqrt1/1 -> Gain2/1  "sqrt(h2)"
  1/pA1/1 -> w_f_inn/pA/1  "w_inn/pA"
  Gain2/1 -> w_ut/1, Sum3/2

== system prosjektoppgave/gamma=0.2alpha/PID ==
  -e'=-(r-h2)'=h2' : Inport
  e : Inport  Port=2
  Gain : Gain  Gain=1.7411
  Gain1 : Gain  Gain=-5.1199
  Gain2 : Gain  Gain=0.1009
  Integrator : Integrator
  Sum : Sum  Inputs=+++
  u : Outport
  wires:
  Integrator/1 -> Gain2/1
  Gain/1 -> Sum/2
  e/1 -> Gain/1, Integrator/1
  Gain2/1 -> Sum/3
  Gain1/1 -> Sum/1
  Sum/1 -> u/1
  -e'=-(r-h2)'=h2'/1 -> Gain1/1

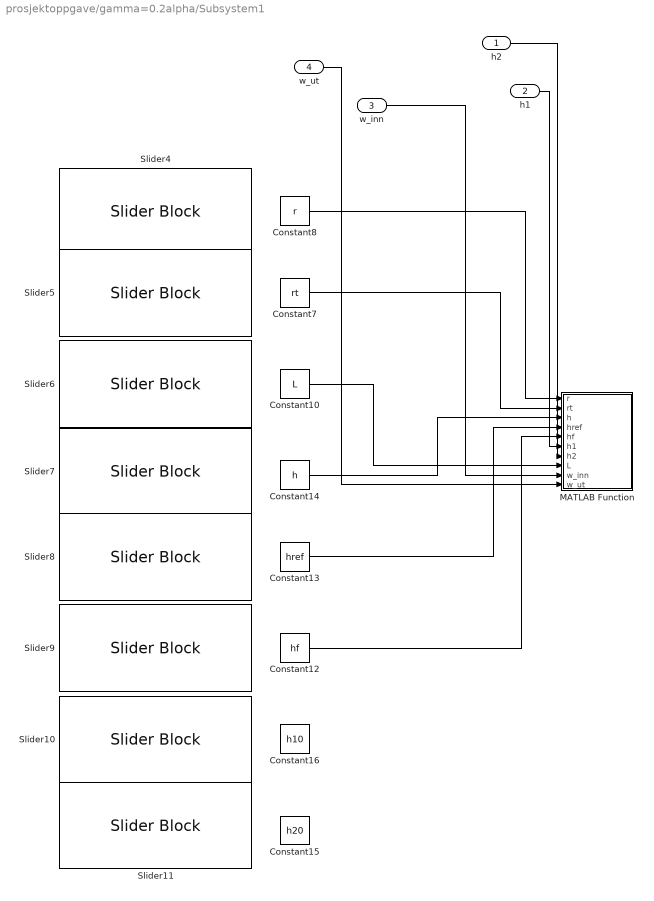
== system prosjektoppgave/gamma=0.2alpha/Subsystem1 ==
  h2 : Inport
  h1 : Inport  Port=2
  w_inn : Inport  Port=3
  w_ut : Inport  Port=4
  Constant10 : Constant  Value=L
  Constant12 : Constant  Value=hf
  Constant13 : Constant  Value=href
  Constant14 : Constant  Value=h
  Constant15 : Constant  Value=h20
  Constant16 : Constant  Value=h10
  Constant7 : Constant  Value=rt
  Constant8 : Constant  Value=r
  MATLAB Function : MATLAB Function  TreatAsAtomicUnit=on
  Slider{4..5,10..11} (4 alike) : SliderBlock
  Slider{6..9} (4 alike) : SliderBlock  ScaleMax=1
  wires:
  h2/1 -> MATLAB Function/7(h2)
  Constant13/1 -> MATLAB Function/4(href)
  Constant10/1 -> MATLAB Function/8(L)
  Constant14/1 -> MATLAB Function/3(h)
  h1/1 -> MATLAB Function/6(h1)
  Constant12/1 -> MATLAB Function/5(hf)
  Constant8/1 -> MATLAB Function/1(r)
  Constant7/1 -> MATLAB Function/2(rt)
  w_inn/1 -> MATLAB Function/9(w_inn)
  w_ut/1 -> MATLAB Function/10(w_ut)

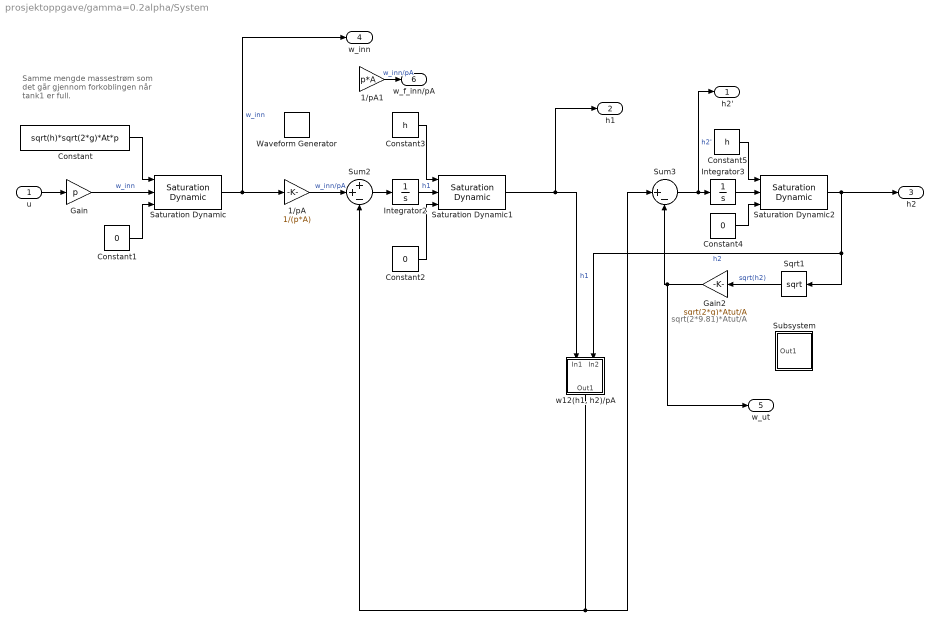
== system prosjektoppgave/gamma=0.2alpha/System ==
  note: Samme mengde massestrøm
      | som det går gjennom
      | forkoblingen når tank1 er full.
  note: sqrt(2*9.81)*Atut/A
  u : Inport  OutMin=0
  1/pA : Gain  Gain=1/(p*A)
  1/pA1 : Gain  Gain=p*A
  Constant : Constant  Value=sqrt(h)*sqrt(2*g)*At*p
  Constant1 : Constant  Value=0
  Constant2 : Constant  Value=0
  Constant3 : Constant  Value=h
  Constant4 : Constant  Value=0
  Constant5 : Constant  Value=h
  Gain : Gain  Gain=p
  Gain2 : Gain  Gain=sqrt(2*g)*Atut/A
  Integrator2 : Integrator  InitialCondition=h10
  Integrator3 : Integrator  InitialCondition=h20
  Saturation Dynamic : sl_discontinuities/Saturation Dynamic  OutMin=[]  OutMax=[]  OutDataTypeStr=Inherit: Same as second input  OutDataType=fixdt(1, 16)  OutScaling=2^-10  DoSatur=off
      settings: LibrarySourceBlock=|
      | simulink/Discontinuities/Saturation
      | Dynamic
  Saturation Dynamic1 : sl_discontinuities/Saturation Dynamic  OutMin=[]  OutMax=[]  OutDataTypeStr=Inherit: Same as second input  OutDataType=fixdt(1, 16)  OutScaling=2^-10  DoSatur=off
      settings: LibrarySourceBlock=|
      | simulink/Discontinuities/Saturation
      | Dynamic
  Saturation Dynamic2 : sl_discontinuities/Saturation Dynamic  OutMin=[]  OutMax=[]  OutDataTypeStr=Inherit: Same as second input  OutDataType=fixdt(1, 16)  OutScaling=2^-10  DoSatur=off
      settings: LibrarySourceBlock=|
      | simulink/Discontinuities/Saturation
      | Dynamic
  Sqrt1 : Sqrt
  Subsystem : Subsystem
  Sum2 : Sum  Inputs=++-
  Sum3 : Sum  Inputs=|+-
  Waveform Generator : simulink/Sources/Waveform Generator  OutMin=0  OutMax=sqrt(2*g)*At/(n*A)  OutDataTypeStr=double  SelectedSignal=1  Signals=sin(sin_Amp, 0.025, 0)  BlockNames=MultiportSwitch_05447e85ab52467  SampleTime=0.1
  "w12(h1, h2)/pA" : Subsystem
  h2' : Outport  VectorParamsAs1DForOutWhenUnconnected=off
  h1 : Outport  Port=2
  h2 : Outport  Port=3
  w_inn : Outport  Port=4
  w_ut : Outport  Port=5
  w_f_inn/pA : Outport  Port=6
  wires:
  Sum2/1 -> Integrator2/1
  Sum3/1 -> h2'/1, Integrator3/1  "h2'"
  Constant1/1 -> Saturation Dynamic/3
  Constant/1 -> Saturation Dynamic/1
  Integrator2/1 -> Saturation Dynamic1/2  "h1"
  Saturation Dynamic1/1 -> "w12(h1, h2)/pA"/1(In1), h1/1  "h1"
  Constant2/1 -> Saturation Dynamic1/3
  Constant3/1 -> Saturation Dynamic1/1
  Integrator3/1 -> Saturation Dynamic2/2
  Saturation Dynamic2/1 -> Sqrt1/1, "w12(h1, h2)/pA"/2(In2), h2/1  "h2"
  Constant4/1 -> Saturation Dynamic2/3
  Constant5/1 -> Saturation Dynamic2/1
  u/1 -> Gain/1
  Gain/1 -> Saturation Dynamic/2  "w_inn"
  Saturation Dynamic/1 -> w_inn/1, 1/pA/1  "w_inn"
  1/pA/1 -> Sum2/2  "w_inn/pA"
  ? -> 1/pA1/1, Sum2/1  "w_f_inn/pA"
  "w12(h1, h2)/pA"/1(Out1) -> Sum3/1, Sum2/3
  Sqrt1/1 -> Gain2/1  "sqrt(h2)"
  1/pA1/1 -> w_f_inn/pA/1  "w_inn/pA"
  Gain2/1 -> w_ut/1, Sum3/2

== system prosjektoppgave/gamma=-0.025alpha/System/Subsystem ==
  Constant1 : Constant  Value=0
  Constant2 : Constant  Value=sqrt(2*g)*Atut*sqrt(h)/A
  Switch : Switch  Threshold=5  SaturateOnIntegerOverflow=off  InputSameDT=off
  Uniform Random Number : UniformRandomNumber  Minimum=0  Maximum=10  SampleTime=20
  Out1 : Outport
  wires:
  Uniform Random Number/1 -> Switch/2
  Switch/1 -> Out1/1
  Constant1/1 -> Switch/1
  Constant2/1 -> Switch/3

== system prosjektoppgave/gamma=-0.025alpha/System/w12(h1, h2)//pA ==
  In1 : Inport
  In2 : Inport  Port=2
  Abs : Abs  SaturateOnIntegerOverflow=off
  Constant8 : Constant  Value=hf
  Gain1 : Gain  Gain=p*At*sqrt(2*g)
  Gain3 : Gain  Gain=1/(p*A)
  Max : MinMax  Function=max  Inputs=2
  Max1 : MinMax  Function=max  Inputs=2
  Product : Product
  Sign : Signum
  Sqrt : Sqrt
  Sum4 : Sum  Inputs=+-
  Out1 : Outport
  wires:
  Constant8/1 -> Max1/2, Max/1
  Sum4/1 -> Sign/1, Abs/1
  Max1/1 -> Sum4/1
  Max/1 -> Sum4/2
  Product/1 -> Gain1/1
  Sqrt/1 -> Product/2
  In1/1 -> Max1/1  "h2"
  Sign/1 -> Product/1
  Abs/1 -> Sqrt/1
  Gain1/1 -> Gain3/1  "w12"
  In2/1 -> Max/2  "h1"
  Gain3/1 -> Out1/1  "w12/pA"

== system prosjektoppgave/gamma=0/System/Subsystem ==
  Constant1 : Constant  Value=0
  Constant2 : Constant  Value=sqrt(2*g)*Atut*sqrt(h)/A
  Switch : Switch  Threshold=5  SaturateOnIntegerOverflow=off  InputSameDT=off
  Uniform Random Number : UniformRandomNumber  Minimum=0  Maximum=10  SampleTime=20
  Out1 : Outport
  wires:
  Uniform Random Number/1 -> Switch/2
  Switch/1 -> Out1/1
  Constant1/1 -> Switch/1
  Constant2/1 -> Switch/3

== system prosjektoppgave/gamma=0/System/w12(h1, h2)//pA ==
  In1 : Inport
  In2 : Inport  Port=2
  Abs : Abs  SaturateOnIntegerOverflow=off
  Constant8 : Constant  Value=hf
  Gain1 : Gain  Gain=p*At*sqrt(2*g)
  Gain3 : Gain  Gain=1/(p*A)
  Max : MinMax  Function=max  Inputs=2
  Max1 : MinMax  Function=max  Inputs=2
  Product : Product
  Sign : Signum
  Sqrt : Sqrt
  Sum4 : Sum  Inputs=+-
  Out1 : Outport
  wires:
  Constant8/1 -> Max1/2, Max/1
  Sum4/1 -> Sign/1, Abs/1
  Max1/1 -> Sum4/1
  Max/1 -> Sum4/2
  Product/1 -> Gain1/1
  Sqrt/1 -> Product/2
  In1/1 -> Max1/1  "h2"
  Sign/1 -> Product/1
  Abs/1 -> Sqrt/1
  Gain1/1 -> Gain3/1  "w12"
  In2/1 -> Max/2  "h1"
  Gain3/1 -> Out1/1  "w12/pA"

== system prosjektoppgave/gamma=0.025alpha/System/Subsystem ==
  Constant1 : Constant  Value=0
  Constant2 : Constant  Value=sqrt(2*g)*Atut*sqrt(h)/A
  Switch : Switch  Threshold=5  SaturateOnIntegerOverflow=off  InputSameDT=off
  Uniform Random Number : UniformRandomNumber  Minimum=0  Maximum=10  SampleTime=20
  Out1 : Outport
  wires:
  Uniform Random Number/1 -> Switch/2
  Switch/1 -> Out1/1
  Constant1/1 -> Switch/1
  Constant2/1 -> Switch/3

== system prosjektoppgave/gamma=0.025alpha/System/w12(h1, h2)//pA ==
  In1 : Inport
  In2 : Inport  Port=2
  Abs : Abs  SaturateOnIntegerOverflow=off
  Constant8 : Constant  Value=hf
  Gain1 : Gain  Gain=p*At*sqrt(2*g)
  Gain3 : Gain  Gain=1/(p*A)
  Max : MinMax  Function=max  Inputs=2
  Max1 : MinMax  Function=max  Inputs=2
  Product : Product
  Sign : Signum
  Sqrt : Sqrt
  Sum4 : Sum  Inputs=+-
  Out1 : Outport
  wires:
  Constant8/1 -> Max1/2, Max/1
  Sum4/1 -> Sign/1, Abs/1
  Max1/1 -> Sum4/1
  Max/1 -> Sum4/2
  Product/1 -> Gain1/1
  Sqrt/1 -> Product/2
  In1/1 -> Max1/1  "h2"
  Sign/1 -> Product/1
  Abs/1 -> Sqrt/1
  Gain1/1 -> Gain3/1  "w12"
  In2/1 -> Max/2  "h1"
  Gain3/1 -> Out1/1  "w12/pA"

== system prosjektoppgave/gamma=0.2alpha/System/Subsystem ==
  Constant1 : Constant  Value=0
  Constant2 : Constant  Value=sqrt(2*g)*Atut*sqrt(h)/A
  Switch : Switch  Threshold=5  SaturateOnIntegerOverflow=off  InputSameDT=off
  Uniform Random Number : UniformRandomNumber  Minimum=0  Maximum=10  SampleTime=20
  Out1 : Outport
  wires:
  Uniform Random Number/1 -> Switch/2
  Switch/1 -> Out1/1
  Constant1/1 -> Switch/1
  Constant2/1 -> Switch/3

== system prosjektoppgave/gamma=0.2alpha/System/w12(h1, h2)//pA ==
  In1 : Inport
  In2 : Inport  Port=2
  Abs : Abs  SaturateOnIntegerOverflow=off
  Constant8 : Constant  Value=hf
  Gain1 : Gain  Gain=p*At*sqrt(2*g)
  Gain3 : Gain  Gain=1/(p*A)
  Max : MinMax  Function=max  Inputs=2
  Max1 : MinMax  Function=max  Inputs=2
  Product : Product
  Sign : Signum
  Sqrt : Sqrt
  Sum4 : Sum  Inputs=+-
  Out1 : Outport
  wires:
  Constant8/1 -> Max1/2, Max/1
  Sum4/1 -> Sign/1, Abs/1
  Max1/1 -> Sum4/1
  Max/1 -> Sum4/2
  Product/1 -> Gain1/1
  Sqrt/1 -> Product/2
  In1/1 -> Max1/1  "h2"
  Sign/1 -> Product/1
  Abs/1 -> Sqrt/1
  Gain1/1 -> Gain3/1  "w12"
  In2/1 -> Max/2  "h1"
  Gain3/1 -> Out1/1  "w12/pA"

== matlab function prosjektoppgave/gamma=0.025alpha/Subsystem1/MATLAB Function ==
  data: r input; rt input; h input; href input; hf input; h1 input; h2 input; L input; w_inn input; w_ut input
function fcn(r, rt, h, href, hf, h1, h2, L, w_inn, w_ut)
    coder.extrinsic('Tank_tegning');
    Tank_tegning(r, rt, h, href, hf, h1, h2, L, w_inn, w_ut);
end

== matlab function prosjektoppgave/gamma=-0.025alpha/Subsystem1/MATLAB Function ==
  data: r input; rt input; h input; href input; hf input; h1 input; h2 input; L input; w_inn input; w_ut input
function fcn(r, rt, h, href, hf, h1, h2, L, w_inn, w_ut)
    coder.extrinsic('Tank_tegning');
    Tank_tegning(r, rt, h, href, hf, h1, h2, L, w_inn, w_ut);
end

== matlab function prosjektoppgave/gamma=0.2alpha/Subsystem1/MATLAB Function ==
  data: r input; rt input; h input; href input; hf input; h1 input; h2 input; L input; w_inn input; w_ut input
function fcn(r, rt, h, href, hf, h1, h2, L, w_inn, w_ut)
    coder.extrinsic('Tank_tegning');
    Tank_tegning(r, rt, h, href, hf, h1, h2, L, w_inn, w_ut);
end

== matlab function prosjektoppgave/gamma=0/Subsystem1/MATLAB Function ==
  data: r input; rt input; h input; href input; hf input; h1 input; h2 input; L input; w_inn input; w_ut input
function fcn(r, rt, h, href, hf, h1, h2, L, w_inn, w_ut)
    coder.extrinsic('Tank_tegning');
    Tank_tegning(r, rt, h, href, hf, h1, h2, L, w_inn, w_ut);
end

== matlab function prosjektoppgave/Subsystem1/MATLAB Function ==
  data: r input; rt input; h input; href input; hf input; h1 input; h2 input; L input; w_inn input; w_ut input
function fcn(r, rt, h, href, hf, h1, h2, L, w_inn, w_ut)
    coder.extrinsic('Tank_tegning');
    Tank_tegning(r, rt, h, href, hf, h1, h2, L, w_inn, w_ut);
end
